simulink subsystem "Propellant_Depletion_Cutoff"  (R2026a)
settings: Solver=VariableStepAuto
settings Model: Creator=asing  LastModifiedBy=asing

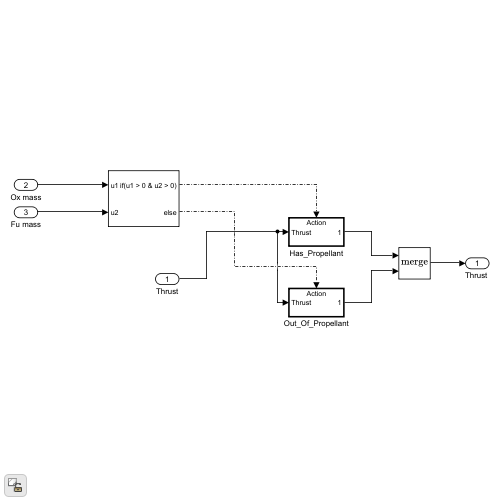
[thumbnail: Simulink's stored preview of the top-level diagram]
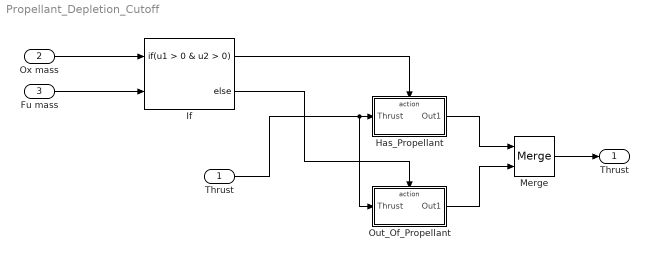
== system Propellant_Depletion_Cutoff ==
  Thrust : Inport
  Ox mass : Inport  Port=2
  Fu mass : Inport  Port=3
  Has_Propellant : Subsystem  TreatAsAtomicUnit=on
  If : If  NumInputs=2  IfExpression=u1 > 0 & u2 > 0
  Merge : Merge
  Out_Of_Propellant : Subsystem  TreatAsAtomicUnit=on
  "Thrust " : Outport
  wires:
  Ox mass/1 -> If/1
  Fu mass/1 -> If/2
  If/1 -> Has_Propellant/Action
  If/2 -> Out_Of_Propellant/Action
  Thrust/1 -> Has_Propellant/1(Thrust), Out_Of_Propellant/1(Thrust)
  Has_Propellant/1(Out1) -> Merge/1
  Out_Of_Propellant/1(Out1) -> Merge/2
  Merge/1 -> "Thrust "/1

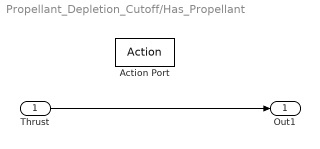
== system Propellant_Depletion_Cutoff/Has_Propellant ==
  Thrust : Inport
  Action Port : ActionPort
  Out1 : Outport
  wires:
  Thrust/1 -> Out1/1

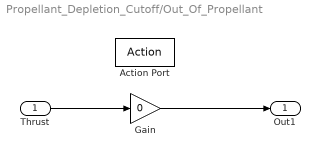
== system Propellant_Depletion_Cutoff/Out_Of_Propellant ==
  Thrust : Inport
  Action Port : ActionPort
  Gain : Gain  Gain=0
  Out1 : Outport
  wires:
  Gain/1 -> Out1/1
  Thrust/1 -> Gain/1
